simulink model "ElectricVehicleThermalManagementWithHeatPump_2026a_version"  (R2026a)
settings: Solver=VariableStepAuto  StopTime=3600  AbsTol=1e-3
PreLoadFcn:
  | init_nmpc
InitFcn:
  | init_nmpc
model workspace: external: MATLAB File ElectricVehicleThermalManagementWithHeatPumpParameters.m (data not in the file)
values from neighbouring files (symbols this model uses):
  battery_C1_LUT = [1913.6 12447 30609 ... (first row only)    [ElectricVehicleThermalManagementWithHeatPumpParameters.m]
  battery_capacity_LUT = [280.081 276.25 276.392]    [ElectricVehicleThermalManagementWithHeatPumpParameters.m]
  battery_cell_cp = 795    [ElectricVehicleThermalManagementWithHeatPumpParameters.m]
  battery_cell_mass = 2.5    [ElectricVehicleThermalManagementWithHeatPumpParameters.m]
  battery_Em_LUT = [3.4966 3.5057 3.5148 ... (first row only)    [ElectricVehicleThermalManagementWithHeatPumpParameters.m]
  battery_N_cells = 20    [ElectricVehicleThermalManagementWithHeatPumpParameters.m]
  battery_Qe_init = 0    [ElectricVehicleThermalManagementWithHeatPumpParameters.m]
  battery_R0_LUT = [0.0117 0.0085 0.009 ... (first row only)    [ElectricVehicleThermalManagementWithHeatPumpParameters.m]
  battery_R1_LUT = [0.0109 0.0029 0.0013 ... (first row only)    [ElectricVehicleThermalManagementWithHeatPumpParameters.m]
  battery_SOC_LUT = [0; 0.1; 0.25; 0.5; 0.75; 0.9; 1]    [ElectricVehicleThermalManagementWithHeatPumpParameters.m]
  battery_T_init = -5    [ElectricVehicleThermalManagementWithHeatPumpParameters.m]
  battery_temperature_LUT = [5 20 40]    [ElectricVehicleThermalManagementWithHeatPumpParameters.m]
  cabin_duct_area = 0.04    [ElectricVehicleThermalManagementWithHeatPumpParameters.m]
  cabin_T_init = -5    [ElectricVehicleThermalManagementWithHeatPumpParameters.m]
  chiller_area_primary = 0.43982297150257105    (= 0.439822971503)    [ElectricVehicleThermalManagementWithHeatPumpParameters.m]
  chiller_N_baffles = 3    [ElectricVehicleThermalManagementWithHeatPumpParameters.m]
  chiller_N_tubes = 100    [ElectricVehicleThermalManagementWithHeatPumpParameters.m]
  chiller_tube_D = 0.0035    [ElectricVehicleThermalManagementWithHeatPumpParameters.m]
  chiller_tube_L = 0.4    [ElectricVehicleThermalManagementWithHeatPumpParameters.m]
  chiller_wall_conductivity = 240    [ElectricVehicleThermalManagementWithHeatPumpParameters.m]
  chiller_wall_thickness = 0.0001    [ElectricVehicleThermalManagementWithHeatPumpParameters.m]
  cond_evap_air_area_flow = 0.3906    [ElectricVehicleThermalManagementWithHeatPumpParameters.m]
  cond_evap_air_area_primary = 1.4834999999999998    (= 1.4835)    [ElectricVehicleThermalManagementWithHeatPumpParameters.m]
  cond_evap_W = 0.015    [ElectricVehicleThermalManagementWithHeatPumpParameters.m]
  cond_evap_wall_conductivity = 240    [ElectricVehicleThermalManagementWithHeatPumpParameters.m]
  cond_evap_wall_thickness = 0.0001    [ElectricVehicleThermalManagementWithHeatPumpParameters.m]
  coolant_channel_D = 0.0092    [ElectricVehicleThermalManagementWithHeatPumpParameters.m]
  coolant_pipe_D = 0.019    [ElectricVehicleThermalManagementWithHeatPumpParameters.m]
  coolant_T_init = -5    [ElectricVehicleThermalManagementWithHeatPumpParameters.m]
  coolant_tank_area = 0.0121    [ElectricVehicleThermalManagementWithHeatPumpParameters.m]
  coolant_tank_volume = 1.25    [ElectricVehicleThermalManagementWithHeatPumpParameters.m]
  coolant_valve_D_ratio_max = 0.95    [ElectricVehicleThermalManagementWithHeatPumpParameters.m]
  coolant_valve_D_ratio_min = 0.001    [ElectricVehicleThermalManagementWithHeatPumpParameters.m]
  coolant_valve_displacement = 0.0063    [ElectricVehicleThermalManagementWithHeatPumpParameters.m]
  coolant_valve_S_max = 0.0053    [ElectricVehicleThermalManagementWithHeatPumpParameters.m]
  evaporator_air_area_flow = 0.12    [ElectricVehicleThermalManagementWithHeatPumpParameters.m]
  evaporator_air_area_primary = 0.4323    [ElectricVehicleThermalManagementWithHeatPumpParameters.m]
  evaporator_W = 0.015    [ElectricVehicleThermalManagementWithHeatPumpParameters.m]
  evaporator_wall_conductivity = 240    [ElectricVehicleThermalManagementWithHeatPumpParameters.m]
  evaporator_wall_thickness = 0.0001    [ElectricVehicleThermalManagementWithHeatPumpParameters.m]
  expansion_valve_D_ratio_max = 0.9    [ElectricVehicleThermalManagementWithHeatPumpParameters.m]
  hex_area_primary = 0.070371675440411369    (= 0.0703716754404)    [ElectricVehicleThermalManagementWithHeatPumpParameters.m]
  hex_N_tubes = 64    [ElectricVehicleThermalManagementWithHeatPumpParameters.m]
  hex_tube_D = 0.0035    [ElectricVehicleThermalManagementWithHeatPumpParameters.m]
  hex_wall_conductivity = 240    [ElectricVehicleThermalManagementWithHeatPumpParameters.m]
  hex_wall_thickness = 0.0001    [ElectricVehicleThermalManagementWithHeatPumpParameters.m]
  inner_cond_air_area_flow = 0.1953    [ElectricVehicleThermalManagementWithHeatPumpParameters.m]
  inner_cond_air_area_primary = 0.99520000000000008    (= 0.9952)    [ElectricVehicleThermalManagementWithHeatPumpParameters.m]
  inner_cond_W = 0.02    [ElectricVehicleThermalManagementWithHeatPumpParameters.m]
  inner_cond_wall_conductivity = 240    [ElectricVehicleThermalManagementWithHeatPumpParameters.m]
  inner_cond_wall_thickness = 0.0001    [ElectricVehicleThermalManagementWithHeatPumpParameters.m]
  pump_speed_max = 1000    [ElectricVehicleThermalManagementWithHeatPumpParameters.m]
  radiator_air_area_flow = 0.097499999999999989    (= 0.0975)    [ElectricVehicleThermalManagementWithHeatPumpParameters.m]
  radiator_air_area_primary = 0.43687499999999996    (= 0.436875)    [ElectricVehicleThermalManagementWithHeatPumpParameters.m]
  radiator_W = 0.015    [ElectricVehicleThermalManagementWithHeatPumpParameters.m]
  radiator_wall_conductivity = 240    [ElectricVehicleThermalManagementWithHeatPumpParameters.m]
  radiator_wall_thickness = 0.0001    [ElectricVehicleThermalManagementWithHeatPumpParameters.m]
  refrigerant_p_init = 0.25    [ElectricVehicleThermalManagementWithHeatPumpParameters.m]
  refrigerant_pipe_D = 0.01    [ElectricVehicleThermalManagementWithHeatPumpParameters.m]
  refrigerant_valve_D_ratio_max = 0.95    [ElectricVehicleThermalManagementWithHeatPumpParameters.m]
  refrigerant_valve_displacement = 0.005    [ElectricVehicleThermalManagementWithHeatPumpParameters.m]
libraries: fl_lib x227, nesl_utility x162, SimscapeFluids_lib x30, LiBatteryElements_lib x16, slpidlib x3, SignalEditorBlockLib x1
(part 8 of 13)

== system ElectricVehicleThermalManagementWithHeatPump_2026a_version/Blower/Recirculation Flap ==
  Max Area [m^2] : Constant  Value=max_area
  Min Area [m^2] : Constant  Value=min_area
  Product : Product
  Restriction AC : fl_lib/Moist Air/Elements/Local Restriction (MA)  restriction_type=foundation.enum.restriction_type.variable  restriction_area=0.001 m^2  min_area=min_area m^2  max_area=max_area m^2  area=port_area m^2  Cd=Cd  B_lam=0.999
  Restriction BC : fl_lib/Moist Air/Elements/Local Restriction (MA)  restriction_type=foundation.enum.restriction_type.variable  restriction_area=0.001 m^2  min_area=min_area m^2  max_area=max_area m^2  area=port_area m^2  Cd=Cd  B_lam=0.999
  Scope : Scope
      settings: ActiveDisplayYMinimum=0.8  ActiveDisplayYMaximum=1  DataLoggingVariableName=ScopeData8
  Simulink-PS Converter : nesl_utility/Simulink-PS Converter  PhysicalDomain=network_engine_domain  SubClassName=ps_input  LeftPortType=input  RightPortType=output  PseudoPeriodic=off  Frequencies=[]  NoiseDistribution=none  NoiseParameters=[]  Unit=m^2  AffineConversion=off  FilteringAndDerivatives=provide  SimscapeFilterOrder=1  InputFilterTimeConstant=0.001  UdotUserProvided=0
  Simulink-PS Converter1 : nesl_utility/Simulink-PS Converter  PhysicalDomain=network_engine_domain  SubClassName=ps_input  LeftPortType=input  RightPortType=output  PseudoPeriodic=off  Frequencies=[]  NoiseDistribution=none  NoiseParameters=[]  Unit=m^2  AffineConversion=off  FilteringAndDerivatives=provide  SimscapeFilterOrder=1  InputFilterTimeConstant=0.001  UdotUserProvided=0
  Sum : Sum  Inputs=+|-
  Sum1 : Sum  Inputs=|+-
  Sum2 : Sum  Inputs=++|
  Transfer Fcn : TransferFcn  Denominator=[tau 1]
  B : PMIOPort  Side=Left
  C : PMIOPort  Port=2  Side=Left
  A : PMIOPort  Port=3  Side=Right
  wires:
  Sum1/1 -> Simulink-PS Converter/1
  Product/1 -> Sum2/1, Sum1/2
  Sum2/1 -> Simulink-PS Converter1/1
  Max Area [m^2]/1 -> Sum/1, Sum1/1
  Min Area [m^2]/1 -> Sum/2, Sum2/2
  Sum/1 -> Product/2
  Transfer Fcn/1 -> Product/1
  [cmd_recirc] -> Scope/1, Transfer Fcn/1
  connections:
  Restriction AC/RConn1 -- Restriction BC/RConn1 -- C/RConn1
  Restriction BC/LConn1 -- B/RConn1
  A/RConn1 -- Restriction AC/LConn1
  Simulink-PS Converter/RConn1 -- Restriction BC/LConn2
  Simulink-PS Converter1/RConn1 -- Restriction AC/LConn2

== system ElectricVehicleThermalManagementWithHeatPump_2026a_version/Cabin/Cabin Heat Transfer ==
  Doors Thermal Mass : fl_lib/Thermal/Thermal Elements/Thermal Mass  mass_type=foundation.enum.constant_variable.constant  mass=doors_mass kg  sp_heat=doors_specific_heat J/kg/K  mass_min=1e-6 kg  num_ports=foundation.enum.numPorts2.two  m_specify=off  m_priority=High  m=1 kg  m_nominal_specify=off  m_nominal_value=1  m_nominal_unit=kg  T_specify=on  T_priority=High  T=doors_initial_temperature degC  T_nominal_specify=off  T_nominal_value=1  T_nominal_unit=K  Q_specify=off  Q_priority=None  Q=0 W  Q_nominal_specify=off  Q_nominal_value=1  Q_nominal_unit=W
  Doors Conduction Inside Half : fl_lib/Thermal/Thermal Elements/Conductive Heat Transfer  thermal_type=foundation.enum.ConstantVariableTabulated.Constant  wall_geometry=foundation.enum.ConductionWallGeometry.Planar  area=doors_area m^2  thickness=doors_thickness / 2 m  d_in=0.05 m  d_out=0.1 m  L=1 m  th_cond_min=10 W/(K*m)  th_cond=doors_conductivity W/(m*K)  th_cond_TLU=[413, 401, 392, 383, 371, 357, 342] W/(K*m)  temp_TLU=[200, 273, 400, 600, 800, 1000, 1200] K  T_specify=off  T_priority=None  T=0 K  T_nominal_specify=off  T_nominal_value=1  T_nominal_unit=K  Q_specify=off  Q_priority=None  Q=0 W  Q_nominal_specify=off  Q_nominal_value=1  Q_nominal_unit=W
  Doors Conduction Outside Half : fl_lib/Thermal/Thermal Elements/Conductive Heat Transfer  thermal_type=foundation.enum.ConstantVariableTabulated.Constant  wall_geometry=foundation.enum.ConductionWallGeometry.Planar  area=doors_area m^2  thickness=doors_thickness / 2 m  d_in=0.05 m  d_out=0.1 m  L=1 m  th_cond_min=10 W/(K*m)  th_cond=doors_conductivity W/(m*K)  th_cond_TLU=[413, 401, 392, 383, 371, 357, 342] W/(K*m)  temp_TLU=[200, 273, 400, 600, 800, 1000, 1200] K  T_specify=off  T_priority=None  T=0 K  T_nominal_specify=off  T_nominal_value=1  T_nominal_unit=K  Q_specify=off  Q_priority=None  Q=0 W  Q_nominal_specify=off  Q_nominal_value=1  Q_nominal_unit=W
  Doors Convection Inside : fl_lib/Thermal/Thermal Elements/Convective Heat Transfer  thermal_type=foundation.enum.constant_variable.constant  area=doors_area m^2  heat_tr_coeff=doors_heat_coeff W/(m^2 * K)  min_heat_tr_coeff=1e-3 W/(K*m^2)  T_specify=off  T_priority=None  T=0 K  T_nominal_specify=off  T_nominal_value=1  T_nominal_unit=K  Q_specify=off  Q_priority=None  Q=0 W  Q_nominal_specify=off  Q_nominal_value=1  Q_nominal_unit=W
  Doors Convection Outside : fl_lib/Thermal/Thermal Elements/Convective Heat Transfer  thermal_type=foundation.enum.constant_variable.constant  area=doors_area m^2  heat_tr_coeff=doors_heat_coeff W/(m^2 * K)  min_heat_tr_coeff=1e-3 W/(K*m^2)  T_specify=off  T_priority=None  T=0 K  T_nominal_specify=off  T_nominal_value=1  T_nominal_unit=K  Q_specify=off  Q_priority=None  Q=0 W  Q_nominal_specify=off  Q_nominal_value=1  Q_nominal_unit=W
  Glass Thermal Mass : fl_lib/Thermal/Thermal Elements/Thermal Mass  mass_type=foundation.enum.constant_variable.constant  mass=glass_mass kg  sp_heat=glass_specific_heat J/kg/K  mass_min=1e-6 kg  num_ports=foundation.enum.numPorts2.two  m_specify=off  m_priority=High  m=1 kg  m_nominal_specify=off  m_nominal_value=1  m_nominal_unit=kg  T_specify=on  T_priority=High  T=glass_initial_temperature degC  T_nominal_specify=off  T_nominal_value=1  T_nominal_unit=K  Q_specify=off  Q_priority=None  Q=0 W  Q_nominal_specify=off  Q_nominal_value=1  Q_nominal_unit=W
  Glass Convection Inside : fl_lib/Thermal/Thermal Elements/Convective Heat Transfer  thermal_type=foundation.enum.constant_variable.constant  area=glass_area m^2  heat_tr_coeff=glass_heat_coeff W/(m^2 * K)  min_heat_tr_coeff=1e-3 W/(K*m^2)  T_specify=off  T_priority=None  T=0 K  T_nominal_specify=off  T_nominal_value=1  T_nominal_unit=K  Q_specify=off  Q_priority=None  Q=0 W  Q_nominal_specify=off  Q_nominal_value=1  Q_nominal_unit=W
  Glass Convection Inside Half : fl_lib/Thermal/Thermal Elements/Conductive Heat Transfer  thermal_type=foundation.enum.ConstantVariableTabulated.Constant  wall_geometry=foundation.enum.ConductionWallGeometry.Planar  area=glass_area m^2  thickness=glass_thickness / 2 m  d_in=0.05 m  d_out=0.1 m  L=1 m  th_cond_min=10 W/(K*m)  th_cond=glass_conductivity W/(m*K)  th_cond_TLU=[413, 401, 392, 383, 371, 357, 342] W/(K*m)  temp_TLU=[200, 273, 400, 600, 800, 1000, 1200] K  T_specify=off  T_priority=None  T=0 K  T_nominal_specify=off  T_nominal_value=1  T_nominal_unit=K  Q_specify=off  Q_priority=None  Q=0 W  Q_nominal_specify=off  Q_nominal_value=1  Q_nominal_unit=W
  Glass Convection Outside : fl_lib/Thermal/Thermal Elements/Convective Heat Transfer  thermal_type=foundation.enum.constant_variable.constant  area=glass_area m^2  heat_tr_coeff=glass_heat_coeff W/(m^2 * K)  min_heat_tr_coeff=1e-3 W/(K*m^2)  T_specify=off  T_priority=None  T=0 K  T_nominal_specify=off  T_nominal_value=1  T_nominal_unit=K  Q_specify=off  Q_priority=None  Q=0 W  Q_nominal_specify=off  Q_nominal_value=1  Q_nominal_unit=W
  Glass Convection Outside Half : fl_lib/Thermal/Thermal Elements/Conductive Heat Transfer  thermal_type=foundation.enum.ConstantVariableTabulated.Constant  wall_geometry=foundation.enum.ConductionWallGeometry.Planar  area=glass_area m^2  thickness=glass_thickness / 2 m  d_in=0.05 m  d_out=0.1 m  L=1 m  th_cond_min=10 W/(K*m)  th_cond=glass_conductivity W/(m*K)  th_cond_TLU=[413, 401, 392, 383, 371, 357, 342] W/(K*m)  temp_TLU=[200, 273, 400, 600, 800, 1000, 1200] K  T_specify=off  T_priority=None  T=0 K  T_nominal_specify=off  T_nominal_value=1  T_nominal_unit=K  Q_specify=off  Q_priority=None  Q=0 W  Q_nominal_specify=off  Q_nominal_value=1  Q_nominal_unit=W
  Roof Thermal Mass : fl_lib/Thermal/Thermal Elements/Thermal Mass  mass_type=foundation.enum.constant_variable.constant  mass=roof_mass kg  sp_heat=roof_specific_heat J/kg/K  mass_min=1e-6 kg  num_ports=foundation.enum.numPorts2.two  m_specify=off  m_priority=High  m=1 kg  m_nominal_specify=off  m_nominal_value=1  m_nominal_unit=kg  T_specify=on  T_priority=High  T=roof_initial_temperature degC  T_nominal_specify=off  T_nominal_value=1  T_nominal_unit=K  Q_specify=off  Q_priority=None  Q=0 W  Q_nominal_specify=off  Q_nominal_value=1  Q_nominal_unit=W
  Roof Conduction Inside Half : fl_lib/Thermal/Thermal Elements/Conductive Heat Transfer  thermal_type=foundation.enum.ConstantVariableTabulated.Constant  wall_geometry=foundation.enum.ConductionWallGeometry.Planar  area=roof_area m^2  thickness=roof_thickness / 2 m  d_in=0.05 m  d_out=0.1 m  L=1 m  th_cond_min=10 W/(K*m)  th_cond=roof_conductivity W/(m*K)  th_cond_TLU=[413, 401, 392, 383, 371, 357, 342] W/(K*m)  temp_TLU=[200, 273, 400, 600, 800, 1000, 1200] K  T_specify=off  T_priority=None  T=0 K  T_nominal_specify=off  T_nominal_value=1  T_nominal_unit=K  Q_specify=off  Q_priority=None  Q=0 W  Q_nominal_specify=off  Q_nominal_value=1  Q_nominal_unit=W
  Roof Conduction Outside Half : fl_lib/Thermal/Thermal Elements/Conductive Heat Transfer  thermal_type=foundation.enum.ConstantVariableTabulated.Constant  wall_geometry=foundation.enum.ConductionWallGeometry.Planar  area=roof_area m^2  thickness=roof_thickness / 2 m  d_in=0.05 m  d_out=0.1 m  L=1 m  th_cond_min=10 W/(K*m)  th_cond=roof_conductivity W/(m*K)  th_cond_TLU=[413, 401, 392, 383, 371, 357, 342] W/(K*m)  temp_TLU=[200, 273, 400, 600, 800, 1000, 1200] K  T_specify=off  T_priority=None  T=0 K  T_nominal_specify=off  T_nominal_value=1  T_nominal_unit=K  Q_specify=off  Q_priority=None  Q=0 W  Q_nominal_specify=off  Q_nominal_value=1  Q_nominal_unit=W
  Roof Convection Inside : fl_lib/Thermal/Thermal Elements/Convective Heat Transfer  thermal_type=foundation.enum.constant_variable.constant  area=roof_area m^2  heat_tr_coeff=roof_heat_coeff W/(m^2 * K)  min_heat_tr_coeff=1e-3 W/(K*m^2)  T_specify=off  T_priority=None  T=0 K  T_nominal_specify=off  T_nominal_value=1  T_nominal_unit=K  Q_specify=off  Q_priority=None  Q=0 W  Q_nominal_specify=off  Q_nominal_value=1  Q_nominal_unit=W
  Roof Convection Outside : fl_lib/Thermal/Thermal Elements/Convective Heat Transfer  thermal_type=foundation.enum.constant_variable.constant  area=roof_area m^2  heat_tr_coeff=roof_heat_coeff W/(m^2 * K)  min_heat_tr_coeff=1e-3 W/(K*m^2)  T_specify=off  T_priority=None  T=0 K  T_nominal_specify=off  T_nominal_value=1  T_nominal_unit=K  Q_specify=off  Q_priority=None  Q=0 W  Q_nominal_specify=off  Q_nominal_value=1  Q_nominal_unit=W
  Inside : PMIOPort  Side=Left
  Outside : PMIOPort  Port=2  Side=Right
  connections:
  Glass Convection Inside/RConn1 -- Glass Convection Inside Half/LConn1
  Glass Convection Outside/LConn1 -- Glass Convection Outside Half/RConn1
  Doors Conduction Outside Half/RConn1 -- Doors Convection Outside/LConn1
  Roof Conduction Outside Half/RConn1 -- Roof Convection Outside/LConn1
  Roof Thermal Mass/LConn1 -- Roof Conduction Inside Half/RConn1
  Glass Thermal Mass/LConn1 -- Glass Convection Inside Half/RConn1
  Doors Convection Inside/RConn1 -- Doors Conduction Inside Half/LConn1
  Doors Convection Outside/RConn1 -- Outside/RConn1 -- Glass Convection Outside/RConn1 -- Roof Convection Outside/RConn1
  Doors Thermal Mass/LConn1 -- Doors Conduction Inside Half/RConn1
  Roof Convection Inside/RConn1 -- Roof Conduction Inside Half/LConn1
  Inside/RConn1 -- Roof Convection Inside/LConn1 -- Doors Convection Inside/LConn1 -- Glass Convection Inside/LConn1
  Glass Thermal Mass/RConn1 -- Glass Convection Outside Half/LConn1
  Doors Thermal Mass/RConn1 -- Doors Conduction Outside Half/LConn1
  Roof Thermal Mass/RConn1 -- Roof Conduction Outside Half/LConn1

== system ElectricVehicleThermalManagementWithHeatPump_2026a_version/Chiller/SR10 ==
  Flow Rate Sensor (2P) : fl_lib/Two-Phase Fluid/Sensors/Flow Rate Sensor (2P)  mass_flow_measure=true  volumetric_flow_measure=false  energy_flow_measure=true
  PS-Simulink Converter : nesl_utility/PS-Simulink Converter  PhysicalDomain=network_engine_domain  SubClassName=ps_output  LeftPortType=input  RightPortType=output  PseudoPeriodic=off  Frequencies=[]  VectorFormat=inherit  Unit=W  AffineConversion=off
  PS-Simulink Converter1 : nesl_utility/PS-Simulink Converter  PhysicalDomain=network_engine_domain  SubClassName=ps_output  LeftPortType=input  RightPortType=output  PseudoPeriodic=off  Frequencies=[]  VectorFormat=inherit  Unit=inherit  AffineConversion=off
  PS-Simulink Converter2 : nesl_utility/PS-Simulink Converter  PhysicalDomain=network_engine_domain  SubClassName=ps_output  LeftPortType=input  RightPortType=output  PseudoPeriodic=off  Frequencies=[]  VectorFormat=inherit  Unit=inherit  AffineConversion=off
  PS-Simulink Converter3 : nesl_utility/PS-Simulink Converter  PhysicalDomain=network_engine_domain  SubClassName=ps_output  LeftPortType=input  RightPortType=output  PseudoPeriodic=off  Frequencies=[]  VectorFormat=inherit  Unit=inherit  AffineConversion=off
  "Pressure, Temperature & Internal Energy Sensor (2P)" : fl_lib/Two-Phase Fluid/Sensors/Pressure, Temperature & Internal Energy Sensor (2P)  reference=foundation.enum.MeasurementReference.absolute  pressure=true  pressure_spec=foundation.enum.PressureMeasementSpec.Absolute  temperature=false  internal_energy=false
  Thermodynamic Properties Sensor (2P) : fl_lib/Two-Phase Fluid/Sensors/Thermodynamic Properties Sensor (2P)  temperature=true  enthalpy=true  density=true  specific_volume=false  entropy=true
  To Workspace : ToWorkspace  VariableName=refChillTemp_out  SampleTime=-1
  To Workspace1 : ToWorkspace  VariableName=refChillH_out  SampleTime=-1
  To Workspace2 : ToWorkspace  VariableName=refChillRho_out  SampleTime=-1
  A : PMIOPort  Side=Left
  B : PMIOPort  Port=2  Side=Right
  tag scope: Phi_chiller_out=global
  wires:
  PS-Simulink Converter/1 -> [Phi_chiller_out]
  PS-Simulink Converter1/1 -> To Workspace/1
  PS-Simulink Converter2/1 -> To Workspace1/1
  PS-Simulink Converter3/1 -> To Workspace2/1
  connections:
  PS-Simulink Converter/LConn1 -- Flow Rate Sensor (2P)/RConn3
  B/RConn1 -- Flow Rate Sensor (2P)/RConn1
  Thermodynamic Properties Sensor (2P)/LConn1 -- A/RConn1 -- "Pressure, Temperature & Internal Energy Sensor (2P)"/LConn1 -- Flow Rate Sensor (2P)/LConn1
  PS-Simulink Converter1/LConn1 -- Thermodynamic Properties Sensor (2P)/RConn1
  Thermodynamic Properties Sensor (2P)/RConn2 -- PS-Simulink Converter2/LConn1
  Thermodynamic Properties Sensor (2P)/RConn3 -- PS-Simulink Converter3/LConn1

== system ElectricVehicleThermalManagementWithHeatPump_2026a_version/Chiller/SR9 ==
  Flow Rate Sensor (2P) : fl_lib/Two-Phase Fluid/Sensors/Flow Rate Sensor (2P)  mass_flow_measure=true  volumetric_flow_measure=false  energy_flow_measure=true
  PS-Simulink Converter : nesl_utility/PS-Simulink Converter  PhysicalDomain=network_engine_domain  SubClassName=ps_output  LeftPortType=input  RightPortType=output  PseudoPeriodic=off  Frequencies=[]  VectorFormat=inherit  Unit=W  AffineConversion=off
  PS-Simulink Converter1 : nesl_utility/PS-Simulink Converter  PhysicalDomain=network_engine_domain  SubClassName=ps_output  LeftPortType=input  RightPortType=output  PseudoPeriodic=off  Frequencies=[]  VectorFormat=inherit  Unit=inherit  AffineConversion=off
  PS-Simulink Converter2 : nesl_utility/PS-Simulink Converter  PhysicalDomain=network_engine_domain  SubClassName=ps_output  LeftPortType=input  RightPortType=output  PseudoPeriodic=off  Frequencies=[]  VectorFormat=inherit  Unit=inherit  AffineConversion=off
  PS-Simulink Converter3 : nesl_utility/PS-Simulink Converter  PhysicalDomain=network_engine_domain  SubClassName=ps_output  LeftPortType=input  RightPortType=output  PseudoPeriodic=off  Frequencies=[]  VectorFormat=inherit  Unit=inherit  AffineConversion=off
  "Pressure, Temperature & Internal Energy Sensor (2P)" : fl_lib/Two-Phase Fluid/Sensors/Pressure, Temperature & Internal Energy Sensor (2P)  reference=foundation.enum.MeasurementReference.absolute  pressure=true  pressure_spec=foundation.enum.PressureMeasementSpec.Absolute  temperature=false  internal_energy=false
  Thermodynamic Properties Sensor (2P) : fl_lib/Two-Phase Fluid/Sensors/Thermodynamic Properties Sensor (2P)  temperature=true  enthalpy=true  density=true  specific_volume=false  entropy=true
  To Workspace : ToWorkspace  VariableName=refChilTemp_in  SampleTime=-1
  To Workspace1 : ToWorkspace  VariableName=refChilH_in  SampleTime=-1
  To Workspace2 : ToWorkspace  VariableName=refChilRho_in  SampleTime=-1
  A : PMIOPort  Side=Left
  B : PMIOPort  Port=2  Side=Right
  tag scope: Phi_chiller_in=global
  wires:
  PS-Simulink Converter/1 -> [Phi_chiller_in]
  PS-Simulink Converter1/1 -> To Workspace/1
  PS-Simulink Converter2/1 -> To Workspace1/1
  PS-Simulink Converter3/1 -> To Workspace2/1
  connections:
  PS-Simulink Converter/LConn1 -- Flow Rate Sensor (2P)/RConn3
  B/RConn1 -- Flow Rate Sensor (2P)/RConn1
  Thermodynamic Properties Sensor (2P)/LConn1 -- A/RConn1 -- "Pressure, Temperature & Internal Energy Sensor (2P)"/LConn1 -- Flow Rate Sensor (2P)/LConn1
  PS-Simulink Converter1/LConn1 -- Thermodynamic Properties Sensor (2P)/RConn1
  Thermodynamic Properties Sensor (2P)/RConn2 -- PS-Simulink Converter2/LConn1
  PS-Simulink Converter3/LConn1 -- Thermodynamic Properties Sensor (2P)/RConn3

== system ElectricVehicleThermalManagementWithHeatPump_2026a_version/Condenser Evaporator/Ram Pressure ==
  1/2 : fl_lib/Physical Signals/Functions/PS Gain  gain=0.5
  PS Product : fl_lib/Physical Signals/Functions/PS Product
  PS-Simulink Converter : nesl_utility/PS-Simulink Converter  PhysicalDomain=network_engine_domain  SubClassName=ps_output  LeftPortType=input  RightPortType=output  PseudoPeriodic=off  Frequencies=[]  VectorFormat=inherit  Unit=inherit  AffineConversion=off
  Pressure Source (MA) : fl_lib/Moist Air/Sources/Pressure Source (MA)  source_type=foundation.enum.constant_controlled.controlled  pressure_differential=0 MPa  power_spec=foundation.enum.power_spec.isentropic  area_A=cabin_duct_area m^2  area_B=cabin_duct_area m^2
  Scope : Scope
      settings: ActiveDisplayYMinimum=-1  ActiveDisplayYMaximum=1  DataLoggingVariableName=ScopeData5
  Thermodynamic Properties Sensor (MA) : fl_lib/Moist Air/Sensors/Thermodynamic Properties Sensor (MA)  measurement_mass_spec=foundation.enum.measurement_mass_spec.mixture  enthalpy=false  enthalpy_reference=foundation.enum.EnthalpyReference.PropertyTables  density=true  specific_heat=false  entropy=false
  sqr : fl_lib/Physical Signals/Functions/PS Math Function  fcn_choice=foundation.enum.math_function.square  v=1
  A : PMIOPort  Side=Left
  V : PMIOPort  Port=2  Side=Left
  B : PMIOPort  Port=3  Side=Right
  wires:
  PS-Simulink Converter/1 -> Scope/1
  connections:
  Pressure Source (MA)/RConn1 -- B/RConn1
  A/RConn1 -- Pressure Source (MA)/LConn1 -- Thermodynamic Properties Sensor (MA)/LConn1
  Pressure Source (MA)/LConn2 -- PS-Simulink Converter/LConn1 -- PS Product/RConn1
  1/2/RConn1 -- PS Product/LConn1
  sqr/RConn1 -- 1/2/LConn1
  V/RConn1 -- sqr/LConn1
  Thermodynamic Properties Sensor (MA)/RConn1 -- PS Product/LConn2

== system ElectricVehicleThermalManagementWithHeatPump_2026a_version/Condenser Evaporator/SR3 ==
  Flow Rate Sensor (2P) : fl_lib/Two-Phase Fluid/Sensors/Flow Rate Sensor (2P)  mass_flow_measure=true  volumetric_flow_measure=false  energy_flow_measure=true
  PS-Simulink Converter : nesl_utility/PS-Simulink Converter  PhysicalDomain=network_engine_domain  SubClassName=ps_output  LeftPortType=input  RightPortType=output  PseudoPeriodic=off  Frequencies=[]  VectorFormat=inherit  Unit=W  AffineConversion=off
  PS-Simulink Converter1 : nesl_utility/PS-Simulink Converter  PhysicalDomain=network_engine_domain  SubClassName=ps_output  LeftPortType=input  RightPortType=output  PseudoPeriodic=off  Frequencies=[]  VectorFormat=inherit  Unit=inherit  AffineConversion=off
  PS-Simulink Converter2 : nesl_utility/PS-Simulink Converter  PhysicalDomain=network_engine_domain  SubClassName=ps_output  LeftPortType=input  RightPortType=output  PseudoPeriodic=off  Frequencies=[]  VectorFormat=inherit  Unit=inherit  AffineConversion=off
  PS-Simulink Converter3 : nesl_utility/PS-Simulink Converter  PhysicalDomain=network_engine_domain  SubClassName=ps_output  LeftPortType=input  RightPortType=output  PseudoPeriodic=off  Frequencies=[]  VectorFormat=inherit  Unit=inherit  AffineConversion=off
  "Pressure, Temperature & Internal Energy Sensor (2P)" : fl_lib/Two-Phase Fluid/Sensors/Pressure, Temperature & Internal Energy Sensor (2P)  reference=foundation.enum.MeasurementReference.absolute  pressure=true  pressure_spec=foundation.enum.PressureMeasementSpec.Absolute  temperature=false  internal_energy=false
  Scope : Scope
      settings: ActiveDisplayYMinimum=247.54122  ActiveDisplayYMaximum=269.48789  DataLoggingVariableName=ScopeData8
  Thermodynamic Properties Sensor (2P) : fl_lib/Two-Phase Fluid/Sensors/Thermodynamic Properties Sensor (2P)  temperature=true  enthalpy=true  density=true  specific_volume=false  entropy=true
  To Workspace : ToWorkspace  VariableName=condEvapRefTemp_inK  SampleTime=-1
  To Workspace1 : ToWorkspace  VariableName=condEvapRefEnthalpy_in  SampleTime=-1
  To Workspace2 : ToWorkspace  VariableName=condEvapRefPress_inMpa  SampleTime=-1
  A : PMIOPort  Side=Left
  B : PMIOPort  Port=2  Side=Right
  tag scope: Phi_cond_evap_in=global
  wires:
  PS-Simulink Converter/1 -> [Phi_cond_evap_in]
  PS-Simulink Converter1/1 -> Scope/1, To Workspace/1
  PS-Simulink Converter2/1 -> To Workspace1/1
  PS-Simulink Converter3/1 -> To Workspace2/1
  connections:
  PS-Simulink Converter/LConn1 -- Flow Rate Sensor (2P)/RConn3
  B/RConn1 -- Flow Rate Sensor (2P)/RConn1
  Thermodynamic Properties Sensor (2P)/LConn1 -- A/RConn1 -- "Pressure, Temperature & Internal Energy Sensor (2P)"/LConn1 -- Flow Rate Sensor (2P)/LConn1
  PS-Simulink Converter1/LConn1 -- Thermodynamic Properties Sensor (2P)/RConn1
  PS-Simulink Converter2/LConn1 -- Thermodynamic Properties Sensor (2P)/RConn2
  PS-Simulink Converter3/LConn1 -- "Pressure, Temperature & Internal Energy Sensor (2P)"/RConn1

== system ElectricVehicleThermalManagementWithHeatPump_2026a_version/Condenser Evaporator/SR4 ==
  Flow Rate Sensor (2P) : fl_lib/Two-Phase Fluid/Sensors/Flow Rate Sensor (2P)  mass_flow_measure=true  volumetric_flow_measure=false  energy_flow_measure=true
  PS-Simulink Converter : nesl_utility/PS-Simulink Converter  PhysicalDomain=network_engine_domain  SubClassName=ps_output  LeftPortType=input  RightPortType=output  PseudoPeriodic=off  Frequencies=[]  VectorFormat=inherit  Unit=W  AffineConversion=off
  PS-Simulink Converter1 : nesl_utility/PS-Simulink Converter  PhysicalDomain=network_engine_domain  SubClassName=ps_output  LeftPortType=input  RightPortType=output  PseudoPeriodic=off  Frequencies=[]  VectorFormat=inherit  Unit=MPa  AffineConversion=off
  PS-Simulink Converter2 : nesl_utility/PS-Simulink Converter  PhysicalDomain=network_engine_domain  SubClassName=ps_output  LeftPortType=input  RightPortType=output  PseudoPeriodic=off  Frequencies=[]  VectorFormat=inherit  Unit=inherit  AffineConversion=off
  PS-Simulink Converter3 : nesl_utility/PS-Simulink Converter  PhysicalDomain=network_engine_domain  SubClassName=ps_output  LeftPortType=input  RightPortType=output  PseudoPeriodic=off  Frequencies=[]  VectorFormat=inherit  Unit=inherit  AffineConversion=off
  "Pressure, Temperature & Internal Energy Sensor (2P)" : fl_lib/Two-Phase Fluid/Sensors/Pressure, Temperature & Internal Energy Sensor (2P)  reference=foundation.enum.MeasurementReference.absolute  pressure=true  pressure_spec=foundation.enum.PressureMeasementSpec.Absolute  temperature=false  internal_energy=false
  Scope : Scope
      settings: ActiveDisplayYMinimum=247.43505  ActiveDisplayYMaximum=269.49229  DataLoggingVariableName=ScopeData9
  Thermodynamic Properties Sensor (2P) : fl_lib/Two-Phase Fluid/Sensors/Thermodynamic Properties Sensor (2P)  temperature=true  enthalpy=true  density=true  specific_volume=false  entropy=true
  To Workspace : ToWorkspace  VariableName=condEvapRefTemp_outK  SampleTime=-1
  To Workspace1 : ToWorkspace  VariableName=condEvapRefEnthaply_out  SampleTime=-1
  To Workspace2 : ToWorkspace  VariableName=condEvapRefPress_outMpa  SampleTime=-1
  A : PMIOPort  Side=Left
  B : PMIOPort  Port=2  Side=Right
  tag scope: Phi_cond_evap_out=global, p_cond_evap_out=global
  wires:
  PS-Simulink Converter/1 -> [Phi_cond_evap_out]
  PS-Simulink Converter1/1 -> To Workspace2/1, [p_cond_evap_out]
  PS-Simulink Converter2/1 -> Scope/1, To Workspace/1
  PS-Simulink Converter3/1 -> To Workspace1/1
  connections:
  PS-Simulink Converter/LConn1 -- Flow Rate Sensor (2P)/RConn3
  B/RConn1 -- Flow Rate Sensor (2P)/RConn1
  Thermodynamic Properties Sensor (2P)/LConn1 -- A/RConn1 -- "Pressure, Temperature & Internal Energy Sensor (2P)"/LConn1 -- Flow Rate Sensor (2P)/LConn1
  PS-Simulink Converter1/LConn1 -- "Pressure, Temperature & Internal Energy Sensor (2P)"/RConn1
  PS-Simulink Converter2/LConn1 -- Thermodynamic Properties Sensor (2P)/RConn1
  Thermodynamic Properties Sensor (2P)/RConn2 -- PS-Simulink Converter3/LConn1

== system ElectricVehicleThermalManagementWithHeatPump_2026a_version/Controls/Battery Heater Control ==
  T_env : Inport
  T_coolant_battery_in : Inport  Port=2
  Constant : Constant  Value=0
  Relay : Relay  OnSwitchValue=15  OffSwitchValue=5  OnOutputValue=0  OffOutputValue=1  ZeroCross=off
  Scope{,1..3} (4 alike) : Scope
      Scope settings: ActiveDisplayYMinimum=-0.125  ActiveDisplayYMaximum=1.125  DataLoggingVariableName=ScopeData4
      Scope1 settings: ActiveDisplayYMinimum=-11  ActiveDisplayYMaximum=-9  DataLoggingVariableName=ScopeData5
      Scope2 settings: ActiveDisplayYMinimum=-15.08835  ActiveDisplayYMaximum=35.79513  DataLoggingVariableName=ScopeData6
      Scope3 settings: ActiveDisplayYMinimum=-0.125  ActiveDisplayYMaximum=1.125  DataLoggingVariableName=ScopeData7
  Switch : Switch  Criteria=u2 > Threshold  Threshold=5  SaturateOnIntegerOverflow=off  InputSameDT=off
  cmd_heater : Outport
  wires:
  T_coolant_battery_in/1 -> Scope2/1, Relay/1
  Switch/1 -> Scope3/1, cmd_heater/1
  T_env/1 -> Scope1/1, Switch/2
  Constant/1 -> Switch/1
  Relay/1 -> Scope/1, Switch/3

== system ElectricVehicleThermalManagementWithHeatPump_2026a_version/Controls/Cabin Air Control ==
  T_cabin : Inport
  T_desired : Inport  Port=2
  T_env : Inport  Port=3
  Blower Control : Subsystem
  Comfort : Subsystem
  Scope : Scope
      settings: ActiveDisplayYMinimum=-0.125  ActiveDisplayYMaximum=1.125  DataLoggingVariableName=ScopeData7
  Scope1 : Scope
      settings: ActiveDisplayYMinimum=9.53499  ActiveDisplayYMaximum=35.09772  DataLoggingVariableName=ScopeData2
  cmd_blower : Outport
  T_cabin_sp : Outport  Port=2
  T_vent_sp : Outport  Port=3
  cmd_recirc : Outport  Port=4
  wires:
  T_cabin/1 -> Comfort/1(T_cabin), Blower Control/1(T_cabin)
  T_desired/1 -> Comfort/2(T_desired)
  T_env/1 -> Blower Control/3(T_env), Comfort/3(T_env)
  Comfort/1(T_cabin_sp) -> T_cabin_sp/1, Blower Control/2(T_cabin_sp)
  Blower Control/1(cmd_blower) -> Scope/1, cmd_blower/1
  Comfort/2(T_vent_sp) -> Scope1/1, T_vent_sp/1
  Comfort/3(cmd_recirc) -> cmd_recirc/1

== system ElectricVehicleThermalManagementWithHeatPump_2026a_version/Controls/Compressor Control ==
  thermal_mode : Inport
  T_vent : Inport  Port=2
  T_vent_sp : Inport  Port=3
  p_low : Inport  Port=4
  p_high : Inport  Port=5
  Constant : Constant  Value=0
  Critical Cutoff : Lookup_n-D  NumberOfTableDimensions=1  BreakpointsForDimension1=[0 3.5 3.6 4]  IndexSearchMethod=Linear search  BeginIndexSearchUsingPreviousIndexResult=on  Table=[1 1 0 0]  ExtrapMethod=Clip  InternalRulePriority=Speed  RndMeth=Simplest
  Freezing Cutoff : Lookup_n-D  NumberOfTableDimensions=1  BreakpointsForDimension1=[0 0.05 0.15 0.3]  IndexSearchMethod=Linear search  BeginIndexSearchUsingPreviousIndexResult=on  Table=[0 0 1 1]  ExtrapMethod=Clip  InternalRulePriority=Speed  RndMeth=Simplest
  PI Controller Cooling : slpidlib/PID Controller  Controller=PI  Form=Parallel  TimeDomain=Continuous-time  UseExternalTs=off  SampleTime=-1  IntegratorMethod=Forward Euler  FilterMethod=Forward Euler  ControllerParametersSource=internal  P=0.05  I=0.005  UseKiTs=off  D=0  UseExternalDerivativeSource=off  N=100  UseFilter=on  TunerSelectOption=Transfer Function Based (PID Tuner App)  ZeroCross=off  InitialConditionSource=internal  InitialConditionForIntegrator=0  InitialConditionForFilter=0  DifferentiatorICPrevScaledInput=0  ExternalReset=either  TrackingMode=off  Kt=1  LimitOutput=on  SatLimitsSource=internal  UpperSaturationLimit=1  LowerSaturationLimit=0  LinearizeAsGain=on  AntiWindupMode=back-calculation  Kb=1  LimitIntegrator=off  UpperIntegratorSaturationLimit=inf  LowerIntegratorSaturationLimit=-inf  POutMin=[]  POutMax=[]  IOutMin=[]  IOutMax=[]  DOutMin=[]  DOutMax=[]  NOutMin=[]  NOutMax=[]  SumOutMin=[]  SumOutMax=[]  SaturationOutMin=[]  SaturationOutMax=[]  PParamMin=[]  PParamMax=[]  IParamMin=[]  IParamMax=[]  DParamMin=[]  DParamMax=[]  NParamMin=[]  NParamMax=[]  KbParamMin=[]  KbParamMax=[]  KtParamMin=[]  KtParamMax=[]  KbOutMin=[]  KbOutMax=[]  KtOutMin=[]  KtOutMax=[]  IntegratorOutMin=[]  IntegratorOutMax=[]  FilterOutMin=[]  FilterOutMax=[]  SumI1OutMin=[]  SumI1OutMax=[]  SumI2OutMin=[]  SumI2OutMax=[]  SumI3OutMin=[]  SumI3OutMax=[]  SumI4OutMin=[]  SumI4OutMax=[]  SumDOutMin=[]  SumDOutMax=[]  DifferentiatorOutMin=[]  DifferentiatorOutMax=[]  FilterDiffOutCoefMin=[]  FilterDiffOutCoefMax=[]  ReciprocalOutMin=[]  ReciprocalOutMax=[]  SumDenOutMin=[]  SumDenOutMax=[]  SumNumOutMin=[]  SumNumOutMax=[]  DivideOutMin=[]  DivideOutMax=[]  UdiffTsProdOutMin=[]  UdiffTsProdOutMax=[]  NTsProdOutMin=[]  NTsProdOutMax=[]  UintegralTsProdOutMin=[]  UintegralTsProdOutMax=[]  UngainTsProdOutMin=[]  UngainTsProdOutMax=[]  ClampingZeroOutDataTypeStr=Inherit: Inherit via back propagation  ClampingZeroOutMin=[]  ClampingZeroOutMax=[]  FilterDenConstantOutDataTypeStr=Inherit: Inherit via back propagation  FilterDenConstantOutMin=[]  FilterDenConstantOutMax=[]  PCopyOutDataTypeStr=Inherit: Inherit via back propagation  PCopyOutMin=[]  PCopyOutMax=[]  NCopyOutDataTypeStr=Inherit: Inherit via back propagation  NCopyOutMin=[]  NCopyOutMax=[]  IntegratorContinuousStateAttributes=''  IntegratorStateMustResolveToSignalObject=off  IntegratorRTWStateStorageClass=Auto  FilterContinuousStateAttributes=''  FilterStateMustResolveToSignalObject=off  FilterRTWStateStorageClass=Auto  ParallelPVariant=InternalParameters  IdealPVariant=Disabled  IVariant=InternalParameters  DVariant=Disabled  IntegratorVariant=Continuous  SatVariant=Enabled  AWVariant=BackCalculation  PCopyVariant=Disabled  TRVariant=Disabled  FdbkBlocksVariant=Forward  IdealPFdbkVariant=Disabled  SatFdbkVariant=Disabled  DerivativeFilterVariant=Disabled  NVariant=Disabled  NCopyVariant=Disabled_SignalSpec  FilterICVariant=Disabled  IntegratorICVariant=InternalICs  ExternalResetVariant=ExternalReset  TRSumVariant=Passthrough  SumFdbkVariant=Disabled  SumVariant=Sum_PI  TsampFilterVariant=InternalTs  TsampNgainVariant=Passthrough  TsampIntegralVariant=Disabled_SignalSpec  ExternalSaturationOutDataTypeStr=Inherit: Same as second input  DerivativeSourceVariant=Disabled  PreIntVariant=InternalPreInt
  PI Controller Heating : slpidlib/PID Controller  Controller=PI  Form=Parallel  TimeDomain=Continuous-time  UseExternalTs=off  SampleTime=-1  IntegratorMethod=Forward Euler  FilterMethod=Forward Euler  ControllerParametersSource=internal  P=-0.05  I=-0.005  UseKiTs=off  D=0  UseExternalDerivativeSource=off  N=100  UseFilter=on  TunerSelectOption=Transfer Function Based (PID Tuner App)  ZeroCross=off  InitialConditionSource=internal  InitialConditionForIntegrator=0  InitialConditionForFilter=0  DifferentiatorICPrevScaledInput=0  ExternalReset=either  TrackingMode=off  Kt=1  LimitOutput=on  SatLimitsSource=internal  UpperSaturationLimit=1  LowerSaturationLimit=0  LinearizeAsGain=on  AntiWindupMode=back-calculation  Kb=1  LimitIntegrator=off  UpperIntegratorSaturationLimit=inf  LowerIntegratorSaturationLimit=-inf  POutMin=[]  POutMax=[]  IOutMin=[]  IOutMax=[]  DOutMin=[]  DOutMax=[]  NOutMin=[]  NOutMax=[]  SumOutMin=[]  SumOutMax=[]  SaturationOutMin=[]  SaturationOutMax=[]  PParamMin=[]  PParamMax=[]  IParamMin=[]  IParamMax=[]  DParamMin=[]  DParamMax=[]  NParamMin=[]  NParamMax=[]  KbParamMin=[]  KbParamMax=[]  KtParamMin=[]  KtParamMax=[]  KbOutMin=[]  KbOutMax=[]  KtOutMin=[]  KtOutMax=[]  IntegratorOutMin=[]  IntegratorOutMax=[]  FilterOutMin=[]  FilterOutMax=[]  SumI1OutMin=[]  SumI1OutMax=[]  SumI2OutMin=[]  SumI2OutMax=[]  SumI3OutMin=[]  SumI3OutMax=[]  SumI4OutMin=[]  SumI4OutMax=[]  SumDOutMin=[]  SumDOutMax=[]  DifferentiatorOutMin=[]  DifferentiatorOutMax=[]  FilterDiffOutCoefMin=[]  FilterDiffOutCoefMax=[]  ReciprocalOutMin=[]  ReciprocalOutMax=[]  SumDenOutMin=[]  SumDenOutMax=[]  SumNumOutMin=[]  SumNumOutMax=[]  DivideOutMin=[]  DivideOutMax=[]  UdiffTsProdOutMin=[]  UdiffTsProdOutMax=[]  NTsProdOutMin=[]  NTsProdOutMax=[]  UintegralTsProdOutMin=[]  UintegralTsProdOutMax=[]  UngainTsProdOutMin=[]  UngainTsProdOutMax=[]  ClampingZeroOutDataTypeStr=Inherit: Inherit via back propagation  ClampingZeroOutMin=[]  ClampingZeroOutMax=[]  FilterDenConstantOutDataTypeStr=Inherit: Inherit via back propagation  FilterDenConstantOutMin=[]  FilterDenConstantOutMax=[]  PCopyOutDataTypeStr=Inherit: Inherit via back propagation  PCopyOutMin=[]  PCopyOutMax=[]  NCopyOutDataTypeStr=Inherit: Inherit via back propagation  NCopyOutMin=[]  NCopyOutMax=[]  IntegratorContinuousStateAttributes=''  IntegratorStateMustResolveToSignalObject=off  IntegratorRTWStateStorageClass=Auto  FilterContinuousStateAttributes=''  FilterStateMustResolveToSignalObject=off  FilterRTWStateStorageClass=Auto  ParallelPVariant=InternalParameters  IdealPVariant=Disabled  IVariant=InternalParameters  DVariant=Disabled  IntegratorVariant=Continuous  SatVariant=Enabled  AWVariant=BackCalculation  PCopyVariant=Disabled  TRVariant=Disabled  FdbkBlocksVariant=Forward  IdealPFdbkVariant=Disabled  SatFdbkVariant=Disabled  DerivativeFilterVariant=Disabled  NVariant=Disabled  NCopyVariant=Disabled_SignalSpec  FilterICVariant=Disabled  IntegratorICVariant=InternalICs  ExternalResetVariant=ExternalReset  TRSumVariant=Passthrough  SumFdbkVariant=Disabled  SumVariant=Sum_PI  TsampFilterVariant=InternalTs  TsampNgainVariant=Passthrough  TsampIntegralVariant=Disabled_SignalSpec  ExternalSaturationOutDataTypeStr=Inherit: Same as second input  DerivativeSourceVariant=Disabled  PreIntVariant=InternalPreInt
  Product : Product
  Product1 : Product
  Scope : Scope
      settings: ActiveDisplayYMinimum=-0.125  ActiveDisplayYMaximum=1.125  DataLoggingVariableName=ScopeData2
  Scope1 : Scope
      settings: ActiveDisplayYMinimum=0.9885  ActiveDisplayYMaximum=1.01925  DataLoggingVariableName=ScopeData3
  Sum : Sum  Inputs=|+-
  Switch : Switch  Criteria=u2 > Threshold  Threshold=1  SaturateOnIntegerOverflow=off  InputSameDT=off
  Switch1 : Switch  Criteria=u2 > Threshold  SaturateOnIntegerOverflow=off  InputSameDT=off
  cmd_comp : Outport
  wires:
  p_low/1 -> Freezing Cutoff/1
  p_high/1 -> Critical Cutoff/1
  T_vent/1 -> Sum/1
  T_vent_sp/1 -> Sum/2
  Sum/1 -> PI Controller Cooling/1, PI Controller Heating/1
  PI Controller Heating/1 -> Switch/1
  PI Controller Cooling/1 -> Switch/3
  Switch1/1 -> cmd_comp/1
  Switch/1 -> Product1/1
  thermal_mode/1 -> Switch1/2, Switch/2, PI Controller Cooling/2, PI Controller Heating/2
  Freezing Cutoff/1 -> Scope1/1, Product/1
  Critical Cutoff/1 -> Scope/1, Product/2
  Product1/1 -> Switch1/1
  Constant/1 -> Switch1/3
  Product/1 -> Product1/2

== system ElectricVehicleThermalManagementWithHeatPump_2026a_version/Controls/Coolant Loop Control ==
  thermal_mode : Inport
  T_env : Inport  Port=2
  T_coolant_inverter_out : Inport  Port=3
  T_motor : Inport  Port=4
  T_battery : Inport  Port=5
  Battery Pump Control : Subsystem
  Motor Pump Control : Subsystem
  Parallel-Serial Mode : Subsystem
  To Workspace : ToWorkspace  VariableName=cmd_parallel_serial  SampleTime=-1
  cmd_parallel_serial : Outport
  cmd_motor_pump : Outport  Port=2
  cmd_battery_pump : Outport  Port=3
  wires:
  Parallel-Serial Mode/1(cmd_parallel_serial) -> To Workspace/1, cmd_parallel_serial/1, Battery Pump Control/3(cmd_parallel_serial)
  Motor Pump Control/1(cmd_motor_pump) -> cmd_motor_pump/1, Battery Pump Control/1(cmd_motor_pump)
  T_env/1 -> Parallel-Serial Mode/2(T_env)
  T_coolant_inverter_out/1 -> Parallel-Serial Mode/3(T_coolant_inverter_out)
  T_motor/1 -> Motor Pump Control/1(T_motor)
  Battery Pump Control/1(cmd_battery_pump) -> cmd_battery_pump/1
  T_battery/1 -> Battery Pump Control/2(T_battery)
  thermal_mode/1 -> Parallel-Serial Mode/1(thermal_mode)

== system ElectricVehicleThermalManagementWithHeatPump_2026a_version/Controls/Fan Control ==
  v_vehicle : Inport
  p_cond : Inport  Port=2
  T_env : Inport  Port=3
  cmd_comp : Inport  Port=4
  T_inverter : Inport  Port=5
  T_motor : Inport  Port=6
  2-D Lookup Table : Lookup_n-D  BreakpointsForDimension1=[0 1 2 3 4]  BreakpointsForDimension2=[0 1 2 3]  BeginIndexSearchUsingPreviousIndexResult=on  Table=[1 2 3 3; 0 1 3 3;0 0 2 3; 0 0 1 3; 0 0 0 3]  ExtrapMethod=Clip  InternalRulePriority=Speed  RndMeth=Simplest
      settings: InputPortMap=u0,u1
  Condenser Requirement : Subsystem
  Constant : Constant  Value=0
  Gain : Gain  Gain=1/3
  Inverter Requirement : Subsystem
  MinMax : MinMax  Function=max  Inputs=3
  Motor Requirement : Subsystem
  Scope{,1..3} (4 alike) : Scope
      Scope settings: ActiveDisplayYMinimum=0.23333  ActiveDisplayYMaximum=0.43333  DataLoggingVariableName=ScopeData14
      Scope1 settings: ActiveDisplayYMinimum=-0.04167  ActiveDisplayYMaximum=0.375  DataLoggingVariableName=ScopeData6
      Scope2 settings: ActiveDisplayYMinimum=-0.04167  ActiveDisplayYMaximum=0.375  DataLoggingVariableName=ScopeData7
      Scope3 settings: ActiveDisplayYMinimum=-0.04167  ActiveDisplayYMaximum=0.375  DataLoggingVariableName=ScopeData8
  Switch : Switch  Criteria=u2 > Threshold  SaturateOnIntegerOverflow=off  InputSameDT=off
  Vehicle Speed Requirement : Subsystem
  cmd_fan : Outport
  wires:
  T_motor/1 -> Motor Requirement/1(T_motor)
  T_inverter/1 -> Inverter Requirement/1(T_inverter)
  p_cond/1 -> Condenser Requirement/1(p_cond)
  T_env/1 -> Condenser Requirement/2(T_env)
  cmd_comp/1 -> Switch/2
  Constant/1 -> Switch/3
  Inverter Requirement/1(cmd_fan) -> Scope3/1, MinMax/2
  Switch/1 -> MinMax/1
  Motor Requirement/1(cmd_fan) -> Scope2/1, MinMax/3
  Vehicle Speed Requirement/1(req) -> 2-D Lookup Table/1
  Condenser Requirement/1(req) -> 2-D Lookup Table/2
  2-D Lookup Table/1 -> Gain/1
  Gain/1 -> Scope/1, Switch/1
  v_vehicle/1 -> Vehicle Speed Requirement/1(v_vehicle)
  MinMax/1 -> Scope1/1, cmd_fan/1
